simulink model "SensorlessHFIFOC"  (R2026b)
settings: Solver=ode4  StopTime=hfiFocTestCfg.Duration  FixedStep=hfiFocTestCfg.PlantStep
PostLoadFcn:
  | addpath(fullfile(fileparts(get_param(bdroot,'FileName')),'..','build_process'));initialize_hfi_foc(bdroot);
model workspace (MAT data in the model file):
  currentCfg.Ts = 5e-05
  currentCfg.BandwidthHz = 500
  currentCfg.Kpd = 3.14159265359
  currentCfg.Kpq = 4.71238898038
  currentCfg.Kid = 1570.79632679
  currentCfg.Kiq = 1570.79632679
  currentCfg.Kaw = 1000
  feedforwardCfg.Enable = 1
  feedforwardCfg.ParameterScale = 1
  focCfg.CurrentMax = 2
  focCfg.Kt = 0.21
  focCfg.FrameCorrectionTolerance = 1e-08
  focCfg.MaxMeasuredCurrent = 8
  focCfg.PositionLossTime = 0.002
  focCfg.PositionLossSamples = 40
  focCfg.SupervisorSettings = [8; 40]
  hfPlantCfg.Rs = 0.5
  hfPlantCfg.Ld = 0.001
  hfPlantCfg.Lq = 0.0015
  hfPlantCfg.Flux = 0.035
  hfPlantCfg.PolePairs = 4
  hfPlantCfg.J = 0.0005
  hfPlantCfg.B = 0.0001
  hfPlantCfg.Id0 = 0
  hfPlantCfg.Iq0 = 0
  hfPlantCfg.Speed0 = 0
  hfPlantCfg.Position0 = 0.175
  hfPlantCfg.SaturationDepth = 0.25
  hfPlantCfg.SaturationCurrent = 1
  hfPlantCfg.CrossInductance = 0
  hfPlantCfg.MechanicalEnabled = 1
  hfPlantCfg.Settings = [0.5; 0.001; 0.0015; 0.035; 4; 0.0005; 0.0001; 0.25; 1; 0; 1]
  hfPlantCfg.InitialState = [0; 0; 0; 0.175]
  hfiCfg.Ts = 5e-05
  hfiCfg.InjectionVoltage = 5
  hfiCfg.Ld = 0.001
  hfiCfg.Lq = 0.0015
  hfiCfg.CrossInductance = 0
  hfiCfg.InitialAxis = 0
  hfiCfg.MaxOmega = 80
  hfiCfg.MinVoltageStep = 1
  hfiCfg.MaxCrossFraction = 0.2
  hfiCfg.MinResponse = 0.01
  hfiCfg.MaxResponse = 0.15
  hfiCfg.MinInjectionScale = 0.1
  hfiCfg.DemodBandwidth = 300
  hfiCfg.DemodFilterEnabled = 1
  hfiCfg.UseMeasuredInverseAverage = 1
  hfiCfg.DemodA = 0.910057240676
  hfiCfg.InverseAverage = 833.333333333
  hfiCfg.CrossPhase = 0
  hfiCfg.InitialTrackerPhase = 0
  hfiCfg.AxisInitialState = [0; 0]
  hfiCfg.DemodSettings = [5e-05; 5; 833.333333333; 0; 1; 0.2; 0.01; 0.15; 0.1; 0.910057240676; 1]
  hfiCfg.TrackSettings = [0; 0; 80]
  hfiFocTestCfg.Ts = 5e-05
  hfiFocTestCfg.PlantStep = 2.5e-06
  hfiFocTestCfg.Duration = 1.2
  hfiFocTestCfg.InitialElectricalAngle = 0.7
  hfiFocTestCfg.InitialElectricalSpeed = 0
  hfiFocTestCfg.SaturationDepth = 0.25
  hfiFocTestCfg.CrossInductance = 0
  hfiFocTestCfg.MechanicalEnabled = 1
  hfiFocTestCfg.Enable = 1
  hfiFocTestCfg.Reset = 0
  hfiFocTestCfg.LoadTorque = 0.02
  hfiFocTestCfg.MeasurementNoise = 0
  hfiFocTestCfg.NoiseSeed = 42
  hfiFocTestCfg.CurrentOffset = [0; 0; 0]
  hfiFocTestCfg.CurrentResolution = 0
  hfiFocTestCfg.CurrentRange = 8
  hfiFocTestCfg.ActuationGain = 1
  hfiFocTestCfg.ExecutionDelay = 0
  hfiFocTestCfg.CurrentDelay = 0
  hfiFocTestCfg.VoltageAlignmentDelay = 0
  hfiFocTestCfg.PulseNegativeGain = 1
  hfiFocTestCfg.PulseFaultOffsetA = 0
  hfiFocTestCfg.QualificationGate = 1
  hfiFocTestCfg.SpeedInitial = 0
  hfiFocTestCfg.SpeedReference = 8
  hfiFocTestCfg.CommandTime = 0.14
  hfiFocTestCfg.TorqueReference = 0.02
  hfiFocTestCfg.Mode = 1
  hfiFocTestCfg.LoadTime = 0.7
  inverterCfg.Vdc = 48
  inverterCfg.MinDuty = 0.02
  inverterCfg.PwmTs = 5e-05
  inverterCfg.LinearLimit = 26.6043004043
  motionCfg.Ts = 0.001
  motionCfg.NaturalFrequency = 20
  motionCfg.Damping = 0.9
  motionCfg.Kt = 0.21
  motionCfg.Kp = 0.0852380952381
  motionCfg.Ki = 0.952380952381
  motionCfg.Kaw = 20
  motionCfg.PositionKp = 8
  motionCfg.SpeedLimit = 15
  motionCfg.AccelerationLimit = 40
  motionCfg.CurrentLimit = 8
  pllCfg.Ts = 5e-05
  pllCfg.NaturalFrequency = 30
  pllCfg.Damping = 0.707
  pllCfg.Kp = 266.532720731
  pllCfg.Ki = 35530.5758439
  pllCfg.Kaw = 376.991118431
  pllCfg.OmegaMax = 160
  pllCfg.MinMagnitude = 0.01
  pllCfg.LockError = 0.12
  pllCfg.LockSamples = 100
  pllCfg.Theta0 = 0
  pllCfg.Omega0 = 0
  pmsmCfg.Rs = 0.5
  pmsmCfg.Ld = 0.001
  pmsmCfg.Lq = 0.0015
  pmsmCfg.Flux = 0.035
  pmsmCfg.PolePairs = 4
  pmsmCfg.J = 0.0005
  pmsmCfg.B = 0.0001
  pmsmCfg.Id0 = 0
  pmsmCfg.Iq0 = 0
  pmsmCfg.Speed0 = 0
  pmsmCfg.Position0 = 0.175
  pmsmCfg.SaturationDepth = 0.25
  pmsmCfg.SaturationCurrent = 1
  pmsmCfg.CrossInductance = 0
  pmsmCfg.MechanicalEnabled = 1
  pmsmCfg.Settings = [0.5; 0.001; 0.0015; 0.035; 4; 0.0005; 0.0001; 0.25; 1; 0; 1]
  pmsmCfg.InitialState = [0; 0; 0; 0.175]
  polarityCfg.Ts = 5e-05
  polarityCfg.PulseVoltage = 4
  polarityCfg.PulseTime = 0.001
  polarityCfg.AxisStableTime = 0.005
  polarityCfg.SettleTime = 0.005
  polarityCfg.DecayStableTime = 0.0005
  polarityCfg.AxisTimeout = 0.2
  polarityCfg.StageTimeout = 0.05
  polarityCfg.TotalTimeout = 0.35
  polarityCfg.CurrentDecay = 0.03
  polarityCfg.MaxCurrent = 6
  polarityCfg.MaxAxisSpeed = 2
  polarityCfg.MinPeakDifference = 0.1
  polarityCfg.MinRelativeDifference = 0.03
  polarityCfg.MinPulseDose = 0.001
  polarityCfg.MaxDoseMismatch = 0.05
  polarityCfg.MaxCrossDoseFraction = 0.1
  polarityCfg.MinPulseVoltage = 0.5
  polarityCfg.SpeedFilterTime = 0.005
  polarityCfg.PulseSamples = 20
  polarityCfg.AxisStableSamples = 100
  polarityCfg.SettleSamples = 100
  polarityCfg.DecayStableSamples = 10
  polarityCfg.AxisTimeoutSamples = 4000
  polarityCfg.StageTimeoutSamples = 1000
  polarityCfg.TotalTimeoutSamples = 7000
  polarityCfg.SpeedA = 0.990049833749
  polarityCfg.Settings = [5e-05; 4; 20; 100; 100; 10; 4000; 1000; 7000; 0.03; 6; 2; 0.1; 0.03; 0.001; 0.05; 0.1; 0.5; 0.990049833749]
  polarityCfg.InitialState = [0; 0; 0; 0; 0; 0; 0; 0; 0; 0; 0; 0; 0; 0; 0; 0; 0; 0; 0]
  probeCfg.Ts = 5e-05
  probeCfg.InjectionVoltage = 5
  probeCfg.WarmupSamples = 32
  probeCfg.CaptureSamples = 256
  probeCfg.MinSaliencyRatio = 0.08
  probeCfg.MaxSaliencyRatio = 0.8
  probeCfg.MinInverseInductance = 100
  probeCfg.MaxInverseInductance = 5000
  probeCfg.MaxFitResidual = 0.2
  probeCfg.MaxAsymmetry = 0.1
  probeCfg.MinVoltageRms = 1
  probeCfg.MaxCurrent = 2
  probeCfg.ProbeAxis = 0
  probeCfg.CrossPhase = 0
  probeCfg.Settings = [5e-05; 5; 32; 256; 0.08; 0.8; 100; 5000; 0.2; 0.1; 1; 2; 0; 0]
  probeCfg.InitialState = [0; 0; 0; 0; 0; 0; 0; 0; 0; 0; 0; 0; 0; 0; 0; 0; 0; 0; 0]
  profileCfg.Ts = 5e-05
  profileCfg.Minimum = -15
  profileCfg.Maximum = 15
  profileCfg.RisingRate = 40
  profileCfg.FallingRate = 40
  profileCfg.RisingStep = 0.002
  profileCfg.FallingStep = 0.002
  refCfg.SpeedTs = 0.001
  refCfg.SpeedKp = 0.0179
  refCfg.SpeedKi = 0.2
  refCfg.SpeedKaw = 20
  testStim.time = [0 5e-05 0.0001 0.00015 0.0002 0.00025 0.0003 0.00035 0.0004 0.00045 0.0005 0.00055 ... (24001 elements, 24001x1)]
  testStim.signals.values = [0 0 0 0 0 0 0 0 0 0 0 0 ... (240010 elements, 24001x10)]
  testStim.signals.dimensions = 10
libraries: ClarkePark x6, HighFrequencyObserver x3, CurrentControl x2, Inverter x2, DQFeedforward x1, CurrentReference x1, MotionControl x1, PMSMHighFrequencyPlant x1
settings Model: Creator=24322  LastModifiedBy=24322

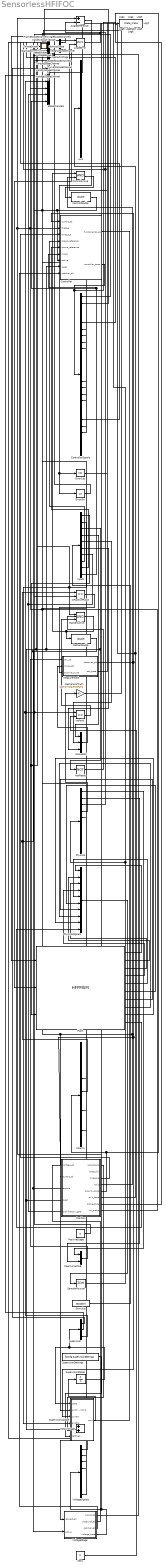
== system SensorlessHFIFOC ==
  AngleDifference : Sum  Inputs=+-
  AngleError : Trigonometry  Operator=atan2
  AngleScope : Scope
  AngleScopeChannels : Mux  Inputs=3
  AppliedVoltage : Demux  Outputs=2
  Axis : Demux  Outputs=15
  ControlActive : Logic  IconShape=distinctive  AllPortsSameDT=off  OutDataTypeStr=boolean
  ControlDouble : DataTypeConversion  OutDataTypeStr=double  SaturateOnIntegerOverflow=off  RndMeth=Floor
  Controller : Subsystem
  ControllerSignals : Demux  Outputs=25
  CurrentScope : Scope
  CurrentScopeChannels : Mux
  ErrorCos : Trigonometry  Operator=cos
  ErrorSin : Trigonometry
  FrameScope : Scope
  FrameScopeChannels : Mux  Inputs=3
  Inputs : Demux  Outputs=10
  IntegralScope : Scope
  IntegralScopeChannels : Mux
  IsPositivePulse : RelationalOperator  Operator===  OutDataTypeStr=boolean  RndMeth=Simplest  InputSameDT=off
  Log1 : ToWorkspace  VariableName=plant_trace  SaveFormat=Structure With Time  SampleTime=hfiCfg.Ts
  Log2 : ToWorkspace  VariableName=probe_trace  SaveFormat=Structure With Time  SampleTime=hfiCfg.Ts
  Log3 : ToWorkspace  VariableName=axis_trace  SaveFormat=Structure With Time  SampleTime=hfiCfg.Ts
  Log4 : ToWorkspace  VariableName=polarity_trace  SaveFormat=Structure With Time  SampleTime=hfiCfg.Ts
  Log5 : ToWorkspace  VariableName=controller_trace  SaveFormat=Structure With Time  SampleTime=hfiCfg.Ts
  Log6 : ToWorkspace  VariableName=voltage_trace  SaveFormat=Structure With Time  SampleTime=hfiCfg.Ts
  Log7 : ToWorkspace  VariableName=adc_trace  SaveFormat=Structure With Time  SampleTime=hfiCfg.Ts
  Log8 : ToWorkspace  VariableName=angle_error  SaveFormat=Structure With Time  SampleTime=hfiCfg.Ts
  LogState : ToWorkspace  VariableName=state_trace  SaveFormat=Structure With Time  SampleTime=hfiCfg.Ts
  MasterActive : Logic  Inputs=3  IconShape=distinctive  AllPortsSameDT=off  OutDataTypeStr=boolean
  MasterDouble : DataTypeConversion  OutDataTypeStr=double  SaturateOnIntegerOverflow=off  RndMeth=Floor
  Measurement : Subsystem
  MechanicalTruth : Gain  Gain=1/pmsmCfg.PolePairs
  NoFault : RelationalOperator  Operator===  OutDataTypeStr=boolean  RndMeth=Simplest  InputSameDT=off
  NoiseABC : Mux  Inputs=3
  NotReset : Logic  Operator=NOT  IconShape=distinctive  AllPortsSameDT=off  OutDataTypeStr=boolean
  Physical : Demux  Outputs=10
  PhysicalSignals : Mux  Inputs=10
  Plant : PMSMHighFrequencyPlant/HFPMSM  cfg=hfPlantCfg
  Polarity : Demux  Outputs=16
  Position : Subsystem
  PositiveStage : Constant  Value=3
  RawCurrentAB : Mux  Inputs=2
  SamplePhysical : ZeroOrderHold  SampleTime=hfiCfg.Ts
  SpeedScope : Scope
  SpeedScopeChannels : Mux  Inputs=3
  StartupScope : Scope
  StartupScopeChannels : Mux
  StateChannels : Mux  Inputs=10
  Stimulus : FromWorkspace  VariableName=testStim  SampleTime=hfiCfg.Ts  Interpolate=off  OutputAfterFinalValue=Holding final value
  Supervisor : Demux  Outputs=3
  SupervisorSettings : Constant  Value=focCfg.SupervisorSettings
  SupervisorStates : UnitDelay  InitialCondition=zeros(3,1)  SampleTime=hfiCfg.Ts
  SupervisorUpdate : MATLAB Function  TreatAsAtomicUnit=on
  TorqueScope : Scope
  TorqueScopeChannels : Mux  Inputs=3
  TotalVoltage : Sum
  ValidityScope : Scope
  ValidityScopeChannels : Mux
  VoltageScope : Scope
  VoltageScopeChannels : Mux  Inputs=5
  VoltageSignals : Demux  Outputs=8
  VoltageStage : Subsystem
  Zero : Constant  Value=0
  wires:
  Stimulus/1 -> Inputs/1
  PhysicalSignals/1 -> SamplePhysical/1
  SamplePhysical/1 -> Log1/1, Physical/1
  RawCurrentAB/1 -> Measurement/1(raw_ab)
  NoiseABC/1 -> Measurement/2(noise_abc)
  IsPositivePulse/1 -> Measurement/3(positive_pulse)
  MasterDouble/1 -> VoltageStage/2(active), Position/3(enable), StateChannels/3
  SupervisorStates/1 -> SupervisorUpdate/1(state), Supervisor/1
  SupervisorSettings/1 -> SupervisorUpdate/6(settings)
  SupervisorUpdate/1(next) -> SupervisorStates/1
  NoFault/1 -> MasterActive/3
  NotReset/1 -> MasterActive/2
  MasterActive/1 -> ControlActive/1, MasterDouble/1
  ControlActive/1 -> ControlDouble/1
  ControlDouble/1 -> ValidityScopeChannels/2, StateChannels/4, Controller/7(active)
  Controller/1(fundamental_ab) -> TotalVoltage/1
  Position/1(request_ab) -> TotalVoltage/2
  TotalVoltage/1 -> VoltageStage/1(request_ab)
  PositiveStage/1 -> IsPositivePulse/2
  AngleDifference/1 -> ErrorCos/1, ErrorSin/1
  ErrorSin/1 -> AngleError/1
  ErrorCos/1 -> AngleError/2
  Inputs/1 -> TorqueScopeChannels/3, Plant/3
  Inputs/2 -> StateChannels/1, SupervisorUpdate/4(enable), MasterActive/1
  Inputs/3 -> StateChannels/2, SupervisorUpdate/5(reset), Position/4(reset), Controller/8(reset), NotReset/1
  Inputs/7 -> Position/5(qualification_gate), StateChannels/9
  Inputs/8 -> Controller/4(speed_reference)
  Inputs/9 -> Controller/5(torque_reference)
  Inputs/10 -> StateChannels/10, Controller/6(mode)
  Supervisor/3 -> ValidityScopeChannels/3, NoFault/1, StateChannels/7
  Zero/1 -> NoFault/2
  Measurement/1(observed_ab) -> SupervisorUpdate/3(current), Position/2(current_ab), Controller/1(current_ab)
  Position/2(theta_full) -> AngleScopeChannels/2, Controller/2(theta_e), AngleDifference/1
  Position/3(omega_e) -> Controller/3(omega_e)
  Position/4(valid) -> ValidityScopeChannels/1, SupervisorUpdate/2(positionValid), ControlActive/2
  Position/5(polarity_trace) -> Polarity/1, Log4/1
  Position/6(axis_trace) -> Log3/1, Axis/1
  Polarity/8 -> StartupScopeChannels/1, IsPositivePulse/1
  Controller/2(controller_trace) -> ControllerSignals/1, Log5/1
  VoltageStage/2(observed_ab) -> Position/1(voltage_ab)
  VoltageStage/3(residual_ab) -> Controller/9(residual_ab)
  VoltageStage/4(voltage_trace) -> VoltageSignals/1, Log6/1
  Physical/3 -> AngleScopeChannels/1, AngleDifference/2
  Physical/4 -> MechanicalTruth/1
  Physical/1 -> RawCurrentAB/1
  Physical/2 -> RawCurrentAB/2
  Inputs/4 -> NoiseABC/1
  Inputs/5 -> NoiseABC/2
  Inputs/6 -> NoiseABC/3
  VoltageStage/1(actual_ab) -> AppliedVoltage/1
  AppliedVoltage/1 -> Plant/1
  AppliedVoltage/2 -> Plant/2
  Plant/1 -> PhysicalSignals/1
  Plant/2 -> PhysicalSignals/2
  Plant/3 -> PhysicalSignals/3
  Plant/4 -> PhysicalSignals/4
  Plant/5 -> PhysicalSignals/5
  Plant/6 -> PhysicalSignals/6
  Plant/7 -> PhysicalSignals/7
  Plant/8 -> PhysicalSignals/8
  Plant/9 -> PhysicalSignals/9
  Plant/10 -> PhysicalSignals/10
  Position/7(probe_trace) -> Log2/1
  Measurement/2(adc_trace) -> Log7/1
  AngleError/1 -> AngleScopeChannels/3, Log8/1
  StateChannels/1 -> LogState/1
  Supervisor/1 -> StateChannels/5
  Supervisor/2 -> StateChannels/6
  Position/8(run_probe) -> StartupScopeChannels/4, StateChannels/8
  SpeedScopeChannels/1 -> SpeedScope/1
  ControllerSignals/1 -> SpeedScopeChannels/1
  MechanicalTruth/1 -> SpeedScopeChannels/2
  ControllerSignals/2 -> SpeedScopeChannels/3
  CurrentScopeChannels/1 -> CurrentScope/1
  ControllerSignals/7 -> CurrentScopeChannels/1
  ControllerSignals/6 -> CurrentScopeChannels/2
  ControllerSignals/8 -> CurrentScopeChannels/3
  ControllerSignals/9 -> CurrentScopeChannels/4
  TorqueScopeChannels/1 -> TorqueScope/1
  ControllerSignals/5 -> TorqueScopeChannels/1
  Physical/5 -> TorqueScopeChannels/2
  AngleScopeChannels/1 -> AngleScope/1
  ValidityScopeChannels/1 -> ValidityScope/1
  Polarity/14 -> ValidityScopeChannels/4
  StartupScopeChannels/1 -> StartupScope/1
  Polarity/6 -> StartupScopeChannels/2
  Polarity/11 -> StartupScopeChannels/3
  VoltageScopeChannels/1 -> VoltageScope/1
  VoltageSignals/1 -> VoltageScopeChannels/1
  VoltageSignals/2 -> VoltageScopeChannels/2
  VoltageSignals/3 -> VoltageScopeChannels/3
  VoltageSignals/4 -> VoltageScopeChannels/4
  VoltageSignals/8 -> VoltageScopeChannels/5
  IntegralScopeChannels/1 -> IntegralScope/1
  ControllerSignals/14 -> IntegralScopeChannels/1
  ControllerSignals/15 -> IntegralScopeChannels/2
  ControllerSignals/16 -> IntegralScopeChannels/3
  ControllerSignals/17 -> IntegralScopeChannels/4
  FrameScopeChannels/1 -> FrameScope/1
  ControllerSignals/20 -> FrameScopeChannels/1
  ControllerSignals/21 -> FrameScopeChannels/2
  ControllerSignals/22 -> FrameScopeChannels/3

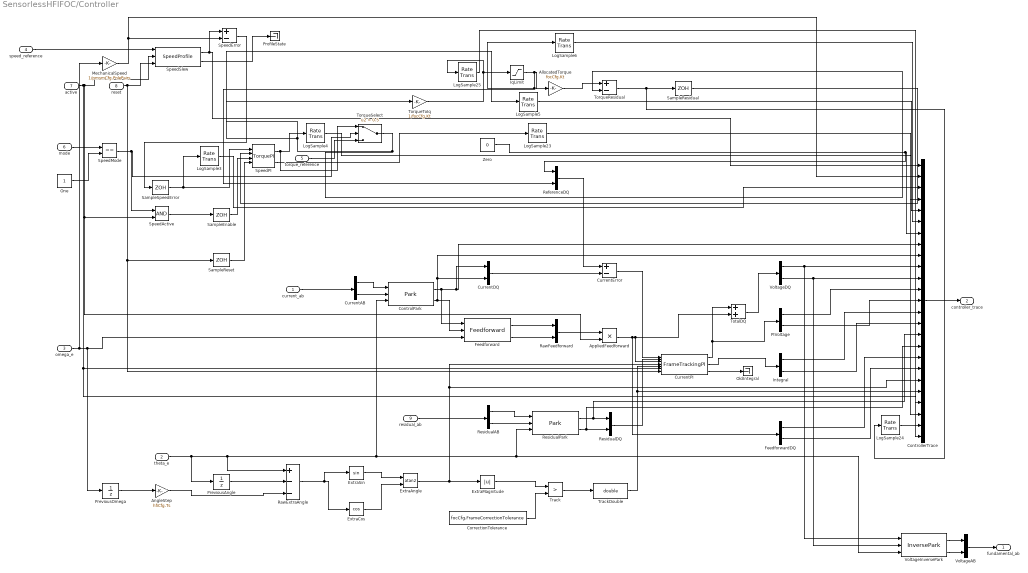
== system SensorlessHFIFOC/Controller ==
  current_ab : Inport
  theta_e : Inport  Port=2
  omega_e : Inport  Port=3
  speed_reference : Inport  Port=4
  torque_reference : Inport  Port=5
  mode : Inport  Port=6
  active : Inport  Port=7
  reset : Inport  Port=8
  residual_ab : Inport  Port=9
  AllocatedTorque : Gain  Gain=focCfg.Kt
  AngleStep : Gain  Gain=hfiCfg.Ts
  AppliedFeedforward : Product  Inputs=**
  ControlPark : ClarkePark/Park  SystemSampleTime=-1  VariantActivationTime=update diagram  EmptyChoice=off  PassThrough=off  PassThroughVariantControl=(default)  EmptyChoiceVariantControl=(default)  AllowFlexibleInterface=on  Latency=0  AutoFrameSizeCalculation=off
  ControllerTrace : Mux  Inputs=25
  CorrectionTolerance : Constant  Value=focCfg.FrameCorrectionTolerance
  CurrentAB : Demux  Outputs=2
  CurrentDQ : Mux  Inputs=2
  CurrentError : Sum  Inputs=+-
  CurrentPI : CurrentControl/FrameTrackingPI  currentCfg=currentCfg
  ExtraAngle : Trigonometry  Operator=atan2
  ExtraCos : Trigonometry  Operator=cos
  ExtraMagnitude : Abs  SaturateOnIntegerOverflow=off
  ExtraSin : Trigonometry
  Feedforward : DQFeedforward/Feedforward  SystemSampleTime=-1  VariantActivationTime=update diagram  EmptyChoice=off  PassThrough=off  PassThroughVariantControl=(default)  EmptyChoiceVariantControl=(default)  AllowFlexibleInterface=on  Latency=0  AutoFrameSizeCalculation=off
  FeedforwardDQ : Demux  Outputs=2
  Integral : Demux  Outputs=2
  IqLimit : Saturate  UpperLimit=focCfg.CurrentMax  LowerLimit=-focCfg.CurrentMax
  LogSample{3..6,23..25} (7 alike) : RateTransition  Integrity=off  Deterministic=off  OutPortSampleTime=hfiCfg.Ts
  MechanicalSpeed : Gain  Gain=1/pmsmCfg.PolePairs
  OldIntegral : Terminator
  One : Constant
  PIVoltage : Demux  Outputs=2
  PreviousAngle : UnitDelay  SampleTime=hfiCfg.Ts
  PreviousOmega : UnitDelay  SampleTime=hfiCfg.Ts
  ProfileState : Terminator
  RawExtraAngle : Sum  Inputs=+--
  RawFeedforward : Mux  Inputs=2
  ReferenceDQ : Mux  Inputs=2
  ResidualAB : Demux  Outputs=2
  ResidualDQ : Mux  Inputs=2
  ResidualPark : ClarkePark/Park  SystemSampleTime=-1  VariantActivationTime=update diagram  EmptyChoice=off  PassThrough=off  PassThroughVariantControl=(default)  EmptyChoiceVariantControl=(default)  AllowFlexibleInterface=on  Latency=0  AutoFrameSizeCalculation=off
  SampleEnable : ZeroOrderHold  SampleTime=refCfg.SpeedTs
  SampleReset : ZeroOrderHold  SampleTime=refCfg.SpeedTs
  SampleResidual : ZeroOrderHold  SampleTime=refCfg.SpeedTs
  SampleSpeedError : ZeroOrderHold  SampleTime=refCfg.SpeedTs
  SpeedActive : Logic  IconShape=distinctive  AllPortsSameDT=off  OutDataTypeStr=boolean
  SpeedError : Sum  Inputs=+-
  SpeedMode : RelationalOperator  Operator===  OutDataTypeStr=boolean  RndMeth=Simplest  InputSameDT=off
  SpeedPI : CurrentReference/TorquePI  SystemSampleTime=-1  VariantActivationTime=update diagram  EmptyChoice=off  PassThrough=off  PassThroughVariantControl=(default)  EmptyChoiceVariantControl=(default)  AllowFlexibleInterface=on  Latency=0  AutoFrameSizeCalculation=off
  SpeedSlew : MotionControl/SpeedProfile  profileCfg=profileCfg
  TorqueResidual : Sum  Inputs=+-
  TorqueSelect : Switch  Criteria=u2 > Threshold  Threshold=0.5  SaturateOnIntegerOverflow=off  InputSameDT=off
  TorqueToIq : Gain  Gain=1/focCfg.Kt
  TotalDQ : Sum
  Track : RelationalOperator  Operator=>  OutDataTypeStr=boolean  RndMeth=Simplest  InputSameDT=off
  TrackDouble : DataTypeConversion  OutDataTypeStr=double  SaturateOnIntegerOverflow=off  RndMeth=Floor
  VoltageAB : Mux  Inputs=2
  VoltageDQ : Demux  Outputs=2
  VoltageInversePark : ClarkePark/InversePark  SystemSampleTime=-1  VariantActivationTime=update diagram  EmptyChoice=off  PassThrough=off  PassThroughVariantControl=(default)  EmptyChoiceVariantControl=(default)  AllowFlexibleInterface=on  Latency=0  AutoFrameSizeCalculation=off
  Zero : Constant  Value=0
  fundamental_ab : Outport
  controller_trace : Outport  Port=2
  wires:
  VoltageInversePark/2 -> VoltageAB/2
  Feedforward/2 -> RawFeedforward/2
  ResidualAB/2 -> ResidualPark/2
  CurrentAB/2 -> ControlPark/2
  VoltageInversePark/1 -> VoltageAB/1
  Feedforward/1 -> RawFeedforward/1
  ResidualAB/1 -> ResidualPark/1
  CurrentAB/1 -> ControlPark/1
  CurrentPI/3 -> OldIntegral/1
  CurrentPI/2 -> Integral/1
  Track/1 -> TrackDouble/1
  CorrectionTolerance/1 -> Track/2
  ExtraMagnitude/1 -> Track/1
  ExtraCos/1 -> ExtraAngle/2
  ExtraSin/1 -> ExtraAngle/1
  RawExtraAngle/1 -> ExtraSin/1, ExtraCos/1
  AngleStep/1 -> RawExtraAngle/3
  PreviousOmega/1 -> AngleStep/1
  PreviousAngle/1 -> RawExtraAngle/2
  ResidualDQ/1 -> CurrentPI/2
  CurrentError/1 -> CurrentPI/1
  CurrentDQ/1 -> CurrentError/2
  ReferenceDQ/1 -> CurrentError/1
  AllocatedTorque/1 -> TorqueResidual/1
  SpeedActive/1 -> SampleEnable/1
  One/1 -> SpeedMode/2
  mode/1 -> SpeedMode/1
  VoltageAB/1 -> fundamental_ab/1
  TotalDQ/1 -> VoltageDQ/1
  CurrentPI/1 -> TotalDQ/1, PIVoltage/1
  AppliedFeedforward/1 -> CurrentPI/3, TotalDQ/2, FeedforwardDQ/1
  RawFeedforward/1 -> AppliedFeedforward/1
  omega_e/1 -> PreviousOmega/1, Feedforward/3, MechanicalSpeed/1
  theta_e/1 -> ResidualPark/3, VoltageInversePark/3, ControlPark/3, RawExtraAngle/1, PreviousAngle/1
  residual_ab/1 -> ResidualAB/1
  current_ab/1 -> CurrentAB/1
  LogSample25/1 -> ControllerTrace/25
  LogSample24/1 -> ControllerTrace/24
  LogSample23/1 -> ControllerTrace/23
  LogSample6/1 -> ControllerTrace/6
  LogSample5/1 -> ControllerTrace/5
  LogSample4/1 -> ControllerTrace/4
  LogSample3/1 -> ControllerTrace/3
  SampleSpeedError/1 -> LogSample3/1, SpeedPI/1
  TorqueResidual/1 -> LogSample24/1, SampleResidual/1
  SampleResidual/1 -> SpeedPI/2
  SpeedMode/1 -> SpeedActive/1, TorqueSelect/2
  SampleEnable/1 -> SpeedPI/3
  SampleReset/1 -> SpeedPI/4
  SpeedPI/1 -> LogSample4/1, TorqueSelect/1
  torque_reference/1 -> TorqueSelect/3
  TorqueSelect/1 -> LogSample5/1, TorqueToIq/1, TorqueResidual/2
  TorqueToIq/1 -> LogSample25/1, IqLimit/1
  IqLimit/1 -> ReferenceDQ/2, LogSample6/1, AllocatedTorque/1
  Zero/1 -> ControllerTrace/7, ReferenceDQ/1
  ExtraAngle/1 -> ControllerTrace/20, CurrentPI/4, ExtraMagnitude/1
  TrackDouble/1 -> CurrentPI/5, ControllerTrace/21
  ControllerTrace/1 -> controller_trace/1
  ControlPark/1 -> ControllerTrace/8, CurrentDQ/1, Feedforward/1
  ControlPark/2 -> ControllerTrace/9, CurrentDQ/2, Feedforward/2
  ResidualPark/1 -> ControllerTrace/16, ResidualDQ/1
  VoltageDQ/1 -> ControllerTrace/10, VoltageInversePark/1
  ResidualPark/2 -> ControllerTrace/17, ResidualDQ/2
  VoltageDQ/2 -> ControllerTrace/11, VoltageInversePark/2
  PIVoltage/1 -> ControllerTrace/12
  PIVoltage/2 -> ControllerTrace/13
  Integral/1 -> ControllerTrace/14
  Integral/2 -> ControllerTrace/15
  FeedforwardDQ/1 -> ControllerTrace/18
  FeedforwardDQ/2 -> ControllerTrace/19
  SpeedPI/2 -> LogSample23/1
  SpeedSlew/2 -> ProfileState/1
  SpeedSlew/1 -> ControllerTrace/1, SpeedError/1
  speed_reference/1 -> SpeedSlew/1
  SpeedError/1 -> SampleSpeedError/1
  MechanicalSpeed/1 -> SpeedError/2, ControllerTrace/2
  active/1 -> ControllerTrace/22, CurrentPI/6, SpeedActive/2, AppliedFeedforward/2, SpeedSlew/2
  reset/1 -> CurrentPI/7, SampleReset/1, SpeedSlew/3

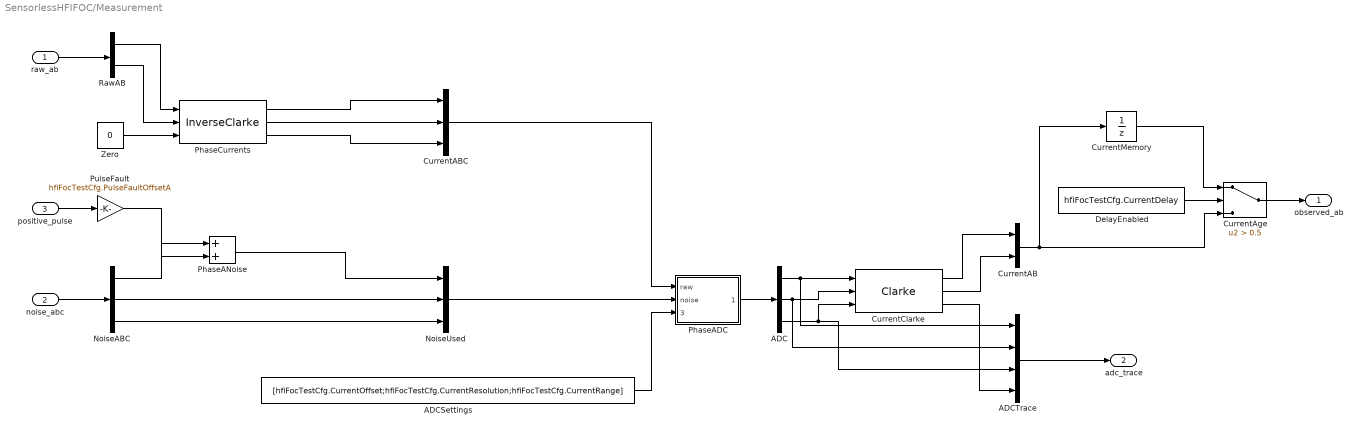
== system SensorlessHFIFOC/Measurement ==
  raw_ab : Inport
  noise_abc : Inport  Port=2
  positive_pulse : Inport  Port=3
  ADC : Demux  Outputs=3
  ADCSettings : Constant  Value=[hfiFocTestCfg.CurrentOffset;hfiFocTestCfg.CurrentResolution;hfiFocTestCfg.CurrentRange]
  ADCTrace : Mux
  CurrentAB : Mux  Inputs=2
  CurrentABC : Mux  Inputs=3
  CurrentAge : Switch  Criteria=u2 > Threshold  Threshold=0.5  SaturateOnIntegerOverflow=off  InputSameDT=off
  CurrentClarke : ClarkePark/Clarke  SystemSampleTime=-1  VariantActivationTime=update diagram  EmptyChoice=off  PassThrough=off  PassThroughVariantControl=(default)  EmptyChoiceVariantControl=(default)  AllowFlexibleInterface=on  Latency=0  AutoFrameSizeCalculation=off
  CurrentMemory : UnitDelay  InitialCondition=zeros(2,1)  SampleTime=hfiCfg.Ts
  DelayEnabled : Constant  Value=hfiFocTestCfg.CurrentDelay
  NoiseABC : Demux  Outputs=3
  NoiseUsed : Mux  Inputs=3
  PhaseADC : MATLAB Function  TreatAsAtomicUnit=on
  PhaseANoise : Sum
  PhaseCurrents : ClarkePark/InverseClarke  SystemSampleTime=-1  VariantActivationTime=update diagram  EmptyChoice=off  PassThrough=off  PassThroughVariantControl=(default)  EmptyChoiceVariantControl=(default)  AllowFlexibleInterface=on  Latency=0  AutoFrameSizeCalculation=off
  PulseFault : Gain  Gain=hfiFocTestCfg.PulseFaultOffsetA
  RawAB : Demux  Outputs=2
  Zero : Constant  Value=0
  observed_ab : Outport
  adc_trace : Outport  Port=2
  wires:
  ADC/3 -> ADCTrace/3, CurrentClarke/3
  PhaseCurrents/3 -> CurrentABC/3
  ADC/2 -> ADCTrace/2, CurrentClarke/2
  PhaseCurrents/2 -> CurrentABC/2
  ADC/1 -> ADCTrace/1, CurrentClarke/1
  PhaseCurrents/1 -> CurrentABC/1
  CurrentClarke/3 -> ADCTrace/4
  CurrentClarke/2 -> CurrentAB/2
  CurrentClarke/1 -> CurrentAB/1
  NoiseABC/3 -> NoiseUsed/3
  NoiseABC/2 -> NoiseUsed/2
  NoiseABC/1 -> PhaseANoise/1
  RawAB/2 -> PhaseCurrents/2
  RawAB/1 -> PhaseCurrents/1
  ADCTrace/1 -> adc_trace/1
  CurrentAge/1 -> observed_ab/1
  DelayEnabled/1 -> CurrentAge/2
  CurrentMemory/1 -> CurrentAge/1
  CurrentAB/1 -> CurrentAge/3, CurrentMemory/1
  Zero/1 -> PhaseCurrents/3
  PhaseADC/1(measured) -> ADC/1
  ADCSettings/1 -> PhaseADC/3(settings)
  CurrentABC/1 -> PhaseADC/1(raw)
  NoiseUsed/1 -> PhaseADC/2(noise)
  PhaseANoise/1 -> NoiseUsed/1
  PulseFault/1 -> PhaseANoise/2
  positive_pulse/1 -> PulseFault/1
  noise_abc/1 -> NoiseABC/1
  raw_ab/1 -> RawAB/1

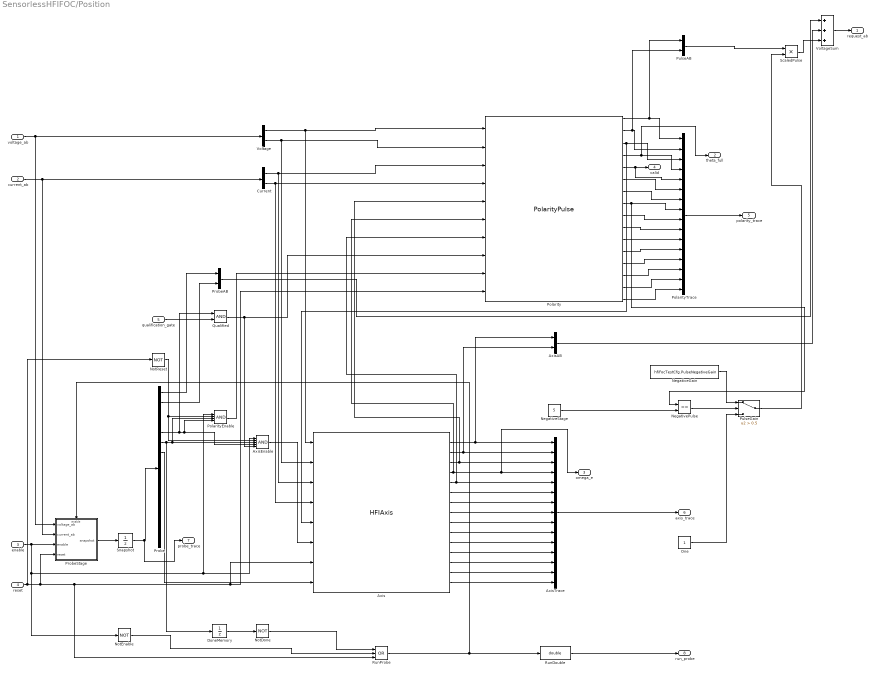
== system SensorlessHFIFOC/Position ==
  voltage_ab : Inport
  current_ab : Inport  Port=2
  enable : Inport  Port=3
  reset : Inport  Port=4
  qualification_gate : Inport  Port=5
  Axis : HighFrequencyObserver/HFIAxis  cfg=hfiCfg  trackerCfg=pllCfg
  AxisAB : Mux  Inputs=2
  AxisEnable : Logic  Inputs=5  IconShape=distinctive  AllPortsSameDT=off  OutDataTypeStr=boolean
  AxisTrace : Mux  Inputs=15
  Current : Demux  Outputs=2
  DoneMemory : UnitDelay  SampleTime=hfiCfg.Ts
  NegativeGain : Constant  Value=hfiFocTestCfg.PulseNegativeGain
  NegativePulse : RelationalOperator  Operator===  OutDataTypeStr=boolean  RndMeth=Simplest  InputSameDT=off
  NegativeStage : Constant  Value=5
  NotDone : Logic  Operator=NOT  IconShape=distinctive  AllPortsSameDT=off  OutDataTypeStr=boolean
  NotEnable : Logic  Operator=NOT  IconShape=distinctive  AllPortsSameDT=off  OutDataTypeStr=boolean
  NotReset : Logic  Operator=NOT  IconShape=distinctive  AllPortsSameDT=off  OutDataTypeStr=boolean
  One : Constant
  Polarity : HighFrequencyObserver/PolarityPulse  cfg=polarityCfg
  PolarityEnable : Logic  Inputs=4  IconShape=distinctive  AllPortsSameDT=off  OutDataTypeStr=boolean
  PolarityTrace : Mux  Inputs=16
  Probe : Demux  Outputs=16
  ProbeAB : Mux  Inputs=2
  ProbeStage : Subsystem
  PulseAB : Mux  Inputs=2
  PulseGain : Switch  Criteria=u2 > Threshold  Threshold=0.5  SaturateOnIntegerOverflow=off  InputSameDT=off
  Qualified : Logic  IconShape=distinctive  AllPortsSameDT=off  OutDataTypeStr=boolean
  RunDouble : DataTypeConversion  OutDataTypeStr=double  SaturateOnIntegerOverflow=off  RndMeth=Floor
  RunProbe : Logic  Operator=OR  Inputs=3  IconShape=distinctive  AllPortsSameDT=off  OutDataTypeStr=boolean
  ScaledPulse : Product  Inputs=**
  Snapshot : UnitDelay  InitialCondition=zeros(16,1)  SampleTime=hfiCfg.Ts
  Voltage : Demux  Outputs=2
  VoltageSum : Sum  Inputs=+++
  request_ab : Outport
  theta_full : Outport  Port=2
  omega_e : Outport  Port=3
  valid : Outport  Port=4
  polarity_trace : Outport  Port=5
  axis_trace : Outport  Port=6
  probe_trace : Outport  Port=7
  run_probe : Outport  Port=8
  wires:
  Polarity/16 -> PolarityTrace/16
  Polarity/15 -> PolarityTrace/15
  Polarity/14 -> PolarityTrace/14
  Polarity/13 -> PolarityTrace/13
  Polarity/12 -> PolarityTrace/12
  Polarity/11 -> PolarityTrace/11
  Polarity/10 -> PolarityTrace/10
  Polarity/9 -> PolarityTrace/9
  Polarity/7 -> PolarityTrace/7
  Polarity/6 -> PolarityTrace/6
  Axis/15 -> AxisTrace/15
  Axis/14 -> AxisTrace/14
  Axis/13 -> AxisTrace/13
  Axis/12 -> AxisTrace/12
  Axis/11 -> AxisTrace/11
  Axis/10 -> AxisTrace/10
  Axis/9 -> AxisTrace/9
  Axis/8 -> AxisTrace/8
  Axis/7 -> AxisTrace/7
  Axis/6 -> AxisTrace/6
  Polarity/2 -> PulseAB/2, PolarityTrace/2
  Axis/2 -> AxisAB/2, AxisTrace/2
  Probe/2 -> ProbeAB/2
  Current/2 -> Axis/4, Polarity/4
  Voltage/2 -> Axis/2, Polarity/2
  Polarity/1 -> PulseAB/1, PolarityTrace/1
  Axis/1 -> AxisAB/1, AxisTrace/1
  Probe/1 -> ProbeAB/1
  Current/1 -> Polarity/3, Axis/3
  Voltage/1 -> Axis/1, Polarity/1
  Polarity/8 -> NegativePulse/1, PolarityTrace/8
  Polarity/5 -> valid/1, PolarityTrace/5
  Polarity/4 -> theta_full/1, PolarityTrace/4
  Polarity/3 -> Axis/5, PolarityTrace/3
  Axis/5 -> Polarity/7, AxisTrace/5
  Axis/4 -> omega_e/1, AxisTrace/4, Polarity/6
  Axis/3 -> Polarity/5, AxisTrace/3
  Probe/7 -> Axis/8
  Probe/5 -> AxisEnable/4, PolarityEnable/4, Qualified/1
  Probe/6 -> AxisEnable/3, PolarityEnable/3, DoneMemory/1
  PulseGain/1 -> ScaledPulse/2
  PulseAB/1 -> ScaledPulse/1
  One/1 -> PulseGain/3
  NegativeGain/1 -> PulseGain/1
  NegativePulse/1 -> PulseGain/2
  NegativeStage/1 -> NegativePulse/2
  VoltageSum/1 -> request_ab/1
  ScaledPulse/1 -> VoltageSum/3
  AxisAB/1 -> VoltageSum/2
  ProbeAB/1 -> VoltageSum/1
  PolarityTrace/1 -> polarity_trace/1
  AxisTrace/1 -> axis_trace/1
  PolarityEnable/1 -> Polarity/9
  AxisEnable/1 -> Axis/6
  Qualified/1 -> AxisEnable/5, Polarity/8
  NotReset/1 -> AxisEnable/2, PolarityEnable/2
  qualification_gate/1 -> Qualified/2
  RunDouble/1 -> run_probe/1
  RunProbe/1 -> ProbeStage/Enable, RunDouble/1
  NotEnable/1 -> RunProbe/2
  NotDone/1 -> RunProbe/1
  DoneMemory/1 -> NotDone/1
  Snapshot/1 -> Probe/1, probe_trace/1
  ProbeStage/1(snapshot) -> Snapshot/1
  reset/1 -> Axis/7, Polarity/10, RunProbe/3, ProbeStage/4(reset), NotReset/1
  enable/1 -> AxisEnable/1, PolarityEnable/1, NotEnable/1, ProbeStage/3(enable)
  current_ab/1 -> ProbeStage/2(current_ab), Current/1
  voltage_ab/1 -> Voltage/1, ProbeStage/1(voltage_ab)

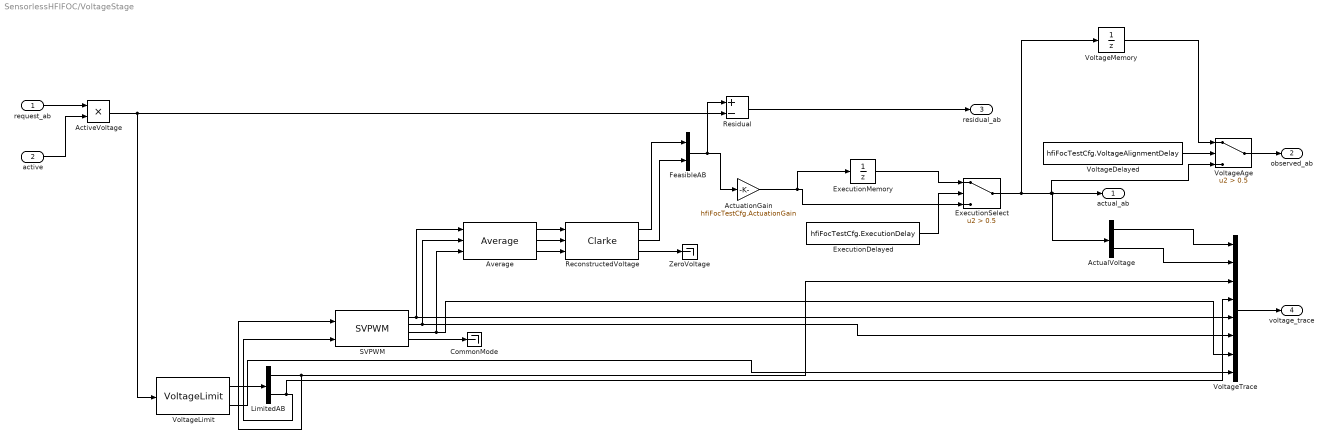
== system SensorlessHFIFOC/VoltageStage ==
  request_ab : Inport
  active : Inport  Port=2
  ActiveVoltage : Product  Inputs=**
  ActualVoltage : Demux  Outputs=2
  ActuationGain : Gain  Gain=hfiFocTestCfg.ActuationGain
  Average : Inverter/Average  SystemSampleTime=-1  VariantActivationTime=update diagram  EmptyChoice=off  PassThrough=off  PassThroughVariantControl=(default)  EmptyChoiceVariantControl=(default)  AllowFlexibleInterface=on  Latency=0  AutoFrameSizeCalculation=off
  CommonMode : Terminator
  ExecutionDelayed : Constant  Value=hfiFocTestCfg.ExecutionDelay
  ExecutionMemory : UnitDelay  InitialCondition=zeros(2,1)  SampleTime=hfiCfg.Ts
  ExecutionSelect : Switch  Criteria=u2 > Threshold  Threshold=0.5  SaturateOnIntegerOverflow=off  InputSameDT=off
  FeasibleAB : Mux  Inputs=2
  LimitedAB : Demux  Outputs=2
  ReconstructedVoltage : ClarkePark/Clarke  SystemSampleTime=-1  VariantActivationTime=update diagram  EmptyChoice=off  PassThrough=off  PassThroughVariantControl=(default)  EmptyChoiceVariantControl=(default)  AllowFlexibleInterface=on  Latency=0  AutoFrameSizeCalculation=off
  Residual : Sum  Inputs=+-
  SVPWM : Inverter/SVPWM  SystemSampleTime=-1  VariantActivationTime=update diagram  EmptyChoice=off  PassThrough=off  PassThroughVariantControl=(default)  EmptyChoiceVariantControl=(default)  AllowFlexibleInterface=on  Latency=0  AutoFrameSizeCalculation=off
  VoltageAge : Switch  Criteria=u2 > Threshold  Threshold=0.5  SaturateOnIntegerOverflow=off  InputSameDT=off
  VoltageDelayed : Constant  Value=hfiFocTestCfg.VoltageAlignmentDelay
  VoltageLimit : CurrentControl/VoltageLimit  SystemSampleTime=-1  VariantActivationTime=update diagram  EmptyChoice=off  PassThrough=off  PassThroughVariantControl=(default)  EmptyChoiceVariantControl=(default)  AllowFlexibleInterface=on  Latency=0  AutoFrameSizeCalculation=off
  VoltageMemory : UnitDelay  InitialCondition=zeros(2,1)  SampleTime=hfiCfg.Ts
  VoltageTrace : Mux  Inputs=8
  ZeroVoltage : Terminator
  actual_ab : Outport
  observed_ab : Outport  Port=2
  residual_ab : Outport  Port=3
  voltage_trace : Outport  Port=4
  wires:
  VoltageLimit/2 -> VoltageTrace/8
  ActualVoltage/2 -> VoltageTrace/2
  ActualVoltage/1 -> VoltageTrace/1
  Average/3 -> ReconstructedVoltage/3
  SVPWM/3 -> Average/3, VoltageTrace/7
  Average/2 -> ReconstructedVoltage/2
  SVPWM/2 -> Average/2, VoltageTrace/6
  Average/1 -> ReconstructedVoltage/1
  SVPWM/1 -> Average/1, VoltageTrace/5
  ReconstructedVoltage/3 -> ZeroVoltage/1
  SVPWM/4 -> CommonMode/1
  LimitedAB/2 -> SVPWM/2, VoltageTrace/4
  LimitedAB/1 -> SVPWM/1, VoltageTrace/3
  VoltageTrace/1 -> voltage_trace/1
  VoltageAge/1 -> observed_ab/1
  VoltageDelayed/1 -> VoltageAge/2
  VoltageMemory/1 -> VoltageAge/1
  ExecutionSelect/1 -> ActualVoltage/1, actual_ab/1, VoltageAge/3, VoltageMemory/1
  ExecutionDelayed/1 -> ExecutionSelect/2
  ExecutionMemory/1 -> ExecutionSelect/1
  ActuationGain/1 -> ExecutionSelect/3, ExecutionMemory/1
  VoltageLimit/1 -> LimitedAB/1
  active/1 -> ActiveVoltage/2
  request_ab/1 -> ActiveVoltage/1
  ActiveVoltage/1 -> Residual/2, VoltageLimit/1
  FeasibleAB/1 -> Residual/1, ActuationGain/1
  Residual/1 -> residual_ab/1
  ReconstructedVoltage/1 -> FeasibleAB/1
  ReconstructedVoltage/2 -> FeasibleAB/2

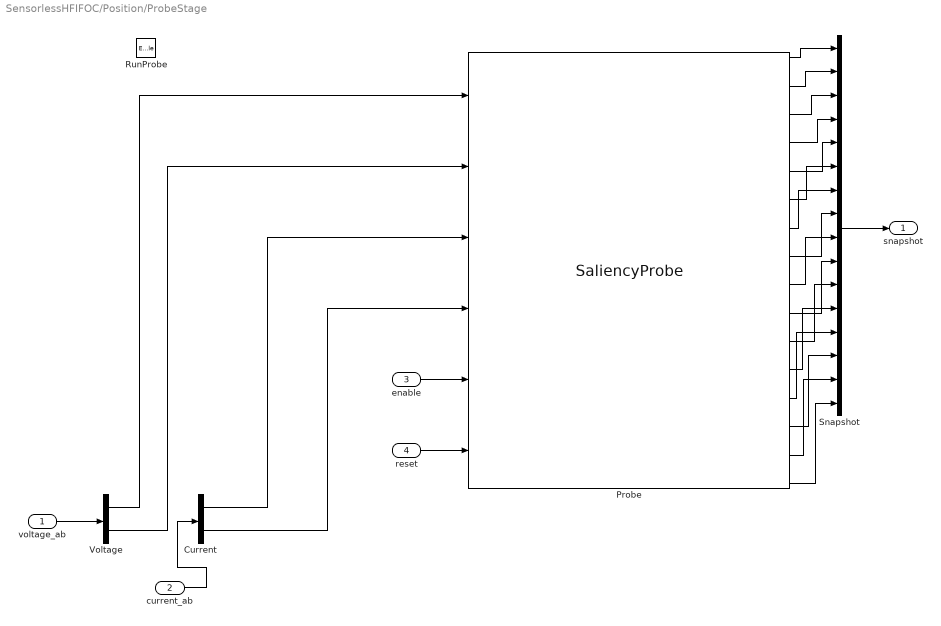
== system SensorlessHFIFOC/Position/ProbeStage ==
  voltage_ab : Inport
  current_ab : Inport  Port=2
  enable : Inport  Port=3
  reset : Inport  Port=4
  RunProbe : EnablePort  StatesWhenEnabling=reset
  Current : Demux  Outputs=2
  Probe : HighFrequencyObserver/SaliencyProbe  cfg=probeCfg
  Snapshot : Mux  Inputs=16
  Voltage : Demux  Outputs=2
  snapshot : Outport  InitialOutput=zeros(16,1)
  wires:
  voltage_ab/1 -> Voltage/1
  current_ab/1 -> Current/1
  enable/1 -> Probe/5
  reset/1 -> Probe/6
  Snapshot/1 -> snapshot/1
  Voltage/1 -> Probe/1
  Current/1 -> Probe/3
  Voltage/2 -> Probe/2
  Current/2 -> Probe/4
  Probe/1 -> Snapshot/1
  Probe/2 -> Snapshot/2
  Probe/3 -> Snapshot/3
  Probe/4 -> Snapshot/4
  Probe/5 -> Snapshot/5
  Probe/6 -> Snapshot/6
  Probe/7 -> Snapshot/7
  Probe/8 -> Snapshot/8
  Probe/9 -> Snapshot/9
  Probe/10 -> Snapshot/10
  Probe/11 -> Snapshot/11
  Probe/12 -> Snapshot/12
  Probe/13 -> Snapshot/13
  Probe/14 -> Snapshot/14
  Probe/15 -> Snapshot/15
  Probe/16 -> Snapshot/16

== matlab function SensorlessHFIFOC/SupervisorUpdate ==
  data: state input; next output; positionValid input; current input; enable input; reset input; settings input
function next=hfi_foc_supervise(state,positionValid,current,enable,reset,settings)
%HFI_FOC_SUPERVISE App-specific held fault; no plant angle or speed is consumed.
% state=[everAcquired;lossSamples;faultCode], fault1=current, fault2=position.
% Output is a separate UnitDelay; this function only prepares the next sample.
%#codegen
next=state;
if enable<.5 || reset>.5,next(:)=0;return;end
if state(3)>.5,return;end
if ~all(isfinite([positionValid;current])) || hypot(current(1),current(2))>settings(1)
    next(3)=1;return;
end
if positionValid>.5,next(1)=1;next(2)=0;
elseif state(1)>.5
    next(2)=state(2)+1;
    if next(2)>=settings(2),next(3)=2;end
end
end

== matlab function SensorlessHFIFOC/Measurement/PhaseADC ==
  data: raw input; measured output; noise input; settings input
function measured=hfi_measure_current(raw,noise,settings)
%HFI_MEASURE_CURRENT Three phase ADC fixture: offset, noise, clipping, rounding.
% settings=[offset_a;offset_b;offset_c;resolution_A;range_A].
%#codegen
measured=min(max(raw+noise+settings(1:3),-settings(5)),settings(5));
if settings(4)>0
    measured=round(measured/settings(4))*settings(4);
end
end
